simulink model "Me492CasterM2V1"  (R2026b)
settings: Solver=ode4  StopTime=4  FixedStep=solver_step_s
InitFcn:
  | addpath(fileparts(fileparts(get_param(bdroot,'FileName')))); m2_model_init(bdroot);
model workspace (MAT data in the model file):
  caster_contact_enabled = 1
  command_sample_dt_s = 0.01
  initial_state = [-0.08; 0; 0; 0; 0; 0; 0; 0; 0; 0; 0; 0; 0]
  p_vector = [16; 0.6; 0.45; 0.0015; 0.0045; 0.00045; -0.08; 0; 0.12; 0.075; 0.38; 0.04; 0.05; -0.18; 0; 9.81; 0.6; 0.6; 300; 600; 200; 250; 0.008; 0.012; 0.00025; 0.0001; 0.004; 0.006; 0.1; 0.08; 0.002; 0.12]
  solver_step_s = 0.0005
  torque_array = [0 0.01 0.02 0.03 0.04 0.05 0.06 0.07 0.08 0.09 0.1 0.11 ... (1203 elements, 401x3)]
settings Model: Creator=lelfs  LastModifiedBy=lelfs
settings DataIOCC: SaveOutput=off  SignalLogging=off

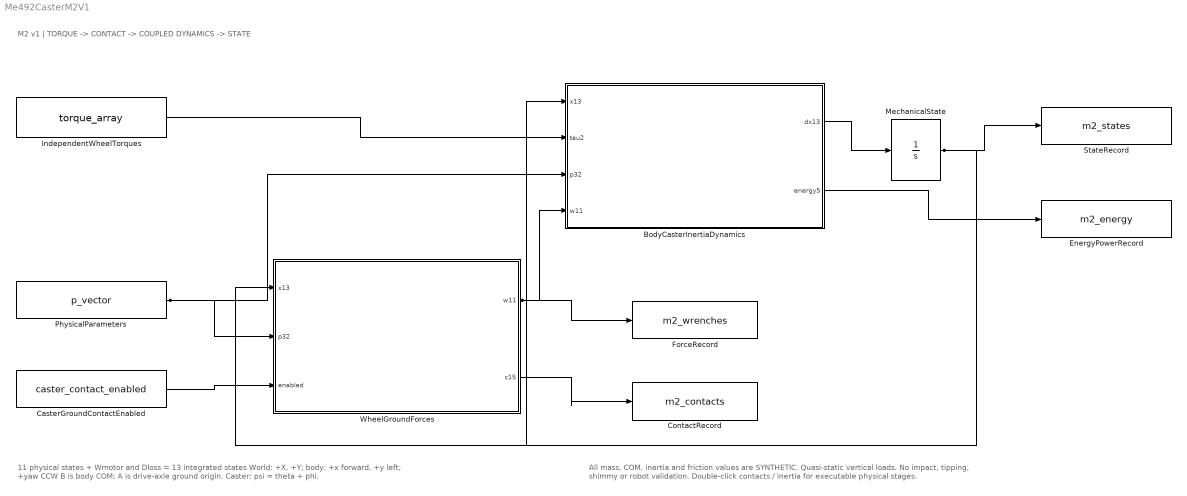
== system Me492CasterM2V1 ==
  note: M2 v1 | TORQUE -> CONTACT -> COUPLED DYNAMICS -> STATE
  note: 11 physical states + Wmotor and Dloss = 13 integrated states
      | World: +X, +Y; body: +x forward, +y left; +yaw CCW
      | B is body COM; A is drive-axle ground origin. Caster: psi = theta + phi.
  note: All mass, COM, inertia and friction values are SYNTHETIC.
      | Quasi-static vertical loads. No impact, tipping, shimmy or robot validation.
      | Double-click contacts / inertia for executable physical stages.
  BodyCasterInertiaDynamics : Subsystem
      mask Display: disp('M * nuDot + bias = Q');port_label('input',1,'x13');port_label('input',2,'tauL/R [N m]');port_label('input',3,'p32 [SI]');port_label('input',4,'F / tau');port_label('output',1,'dx13/dt');port_label('output',2,'energy / power');
  CasterGroundContactEnabled : Constant  Value=caster_contact_enabled
  ContactRecord : ToWorkspace  VariableName=m2_contacts  SaveFormat=Timeseries  SampleTime=-1
  EnergyPowerRecord : ToWorkspace  VariableName=m2_energy  SaveFormat=Timeseries  SampleTime=-1
  ForceRecord : ToWorkspace  VariableName=m2_wrenches  SaveFormat=Timeseries  SampleTime=-1
  IndependentWheelTorques : FromWorkspace  VariableName=torque_array  SampleTime=command_sample_dt_s  Interpolate=off  OutputAfterFinalValue=Holding final value
  MechanicalState : Integrator  InitialCondition=initial_state
  PhysicalParameters : Constant  Value=p_vector
  StateRecord : ToWorkspace  VariableName=m2_states  SaveFormat=Timeseries  SampleTime=-1
  WheelGroundForces : Subsystem
      mask Display: disp('Loads -> slip -> passive contact');port_label('input',1,'x13');port_label('input',2,'p32 [SI]');port_label('input',3,'enabled');port_label('output',1,'F / tau');port_label('output',2,'slip / N');
  wires:
  IndependentWheelTorques/1 -> BodyCasterInertiaDynamics/2(tau2)
  PhysicalParameters/1 -> WheelGroundForces/2(p32), BodyCasterInertiaDynamics/3(p32)
  CasterGroundContactEnabled/1 -> WheelGroundForces/3(enabled)
  WheelGroundForces/1(w11) -> BodyCasterInertiaDynamics/4(w11), ForceRecord/1
  BodyCasterInertiaDynamics/1(dx13) -> MechanicalState/1
  MechanicalState/1 -> StateRecord/1, WheelGroundForces/1(x13), BodyCasterInertiaDynamics/1(x13)
  BodyCasterInertiaDynamics/2(energy5) -> EnergyPowerRecord/1
  WheelGroundForces/2(c15) -> ContactRecord/1

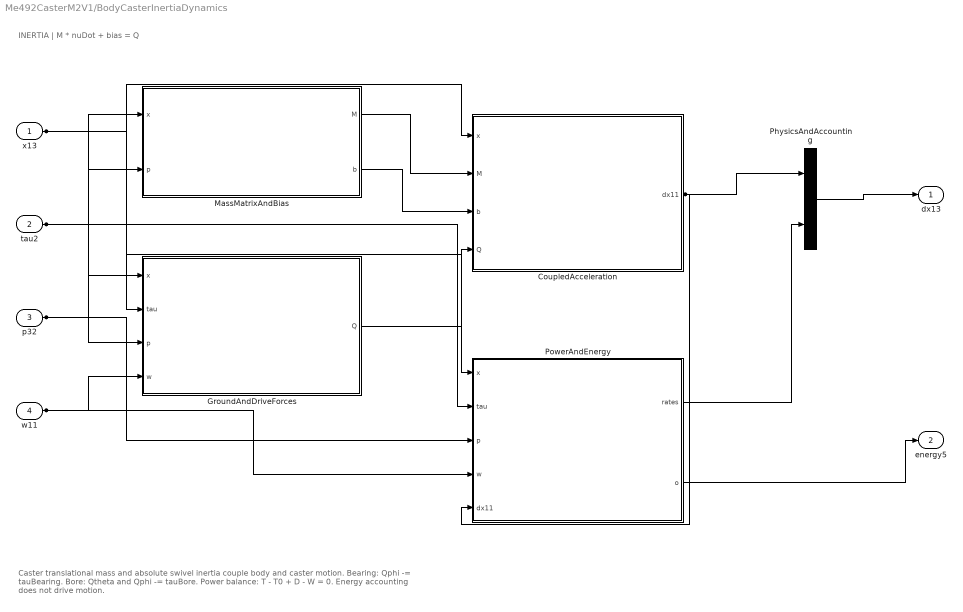
== system Me492CasterM2V1/BodyCasterInertiaDynamics ==
  note: INERTIA | M * nuDot + bias = Q
  note: Caster translational mass and absolute swivel inertia couple body and caster motion.
      | Bearing: Qphi -= tauBearing. Bore: Qtheta and Qphi -= tauBore.
      | Power balance: T - T0 + D - W = 0. Energy accounting does not drive motion.
  x13 : Inport
  tau2 : Inport  Port=2
  p32 : Inport  Port=3
  w11 : Inport  Port=4
  CoupledAcceleration : MATLAB Function  TreatAsAtomicUnit=on
  GroundAndDriveForces : MATLAB Function  TreatAsAtomicUnit=on
  MassMatrixAndBias : MATLAB Function  TreatAsAtomicUnit=on
  PhysicsAndAccounting : Mux  Inputs=2
  PowerAndEnergy : MATLAB Function  TreatAsAtomicUnit=on
  dx13 : Outport
  energy5 : Outport  Port=2
  wires:
  x13/1 -> MassMatrixAndBias/1(x), GroundAndDriveForces/1(x), PowerAndEnergy/1(x), CoupledAcceleration/1(x)
  p32/1 -> MassMatrixAndBias/2(p), GroundAndDriveForces/3(p), PowerAndEnergy/3(p)
  tau2/1 -> GroundAndDriveForces/2(tau), PowerAndEnergy/2(tau)
  w11/1 -> GroundAndDriveForces/4(w), PowerAndEnergy/4(w)
  MassMatrixAndBias/1(M) -> CoupledAcceleration/2(M)
  MassMatrixAndBias/2(b) -> CoupledAcceleration/3(b)
  GroundAndDriveForces/1(Q) -> CoupledAcceleration/4(Q)
  CoupledAcceleration/1(dx11) -> PowerAndEnergy/5(dx11), PhysicsAndAccounting/1
  PowerAndEnergy/1(rates) -> PhysicsAndAccounting/2
  PhysicsAndAccounting/1 -> dx13/1
  PowerAndEnergy/2(o) -> energy5/1

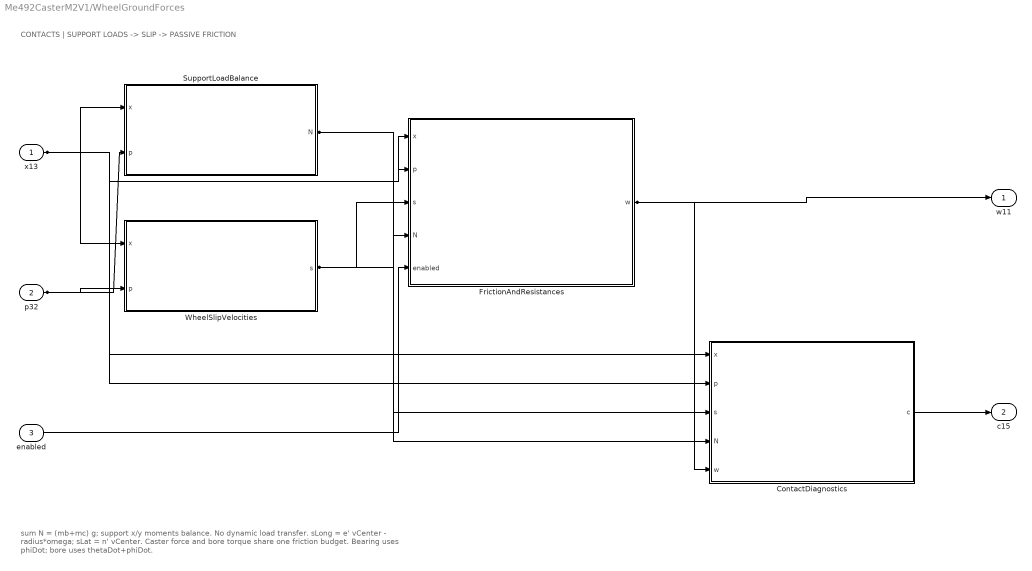
== system Me492CasterM2V1/WheelGroundForces ==
  note: CONTACTS | SUPPORT LOADS -> SLIP -> PASSIVE FRICTION
  note: sum N = (mb+mc) g; support x/y moments balance. No dynamic load transfer.
      | sLong = e' vCenter - radius*omega; sLat = n' vCenter.
      | Caster force and bore torque share one friction budget. Bearing uses phiDot; bore uses thetaDot+phiDot.
  x13 : Inport
  p32 : Inport  Port=2
  enabled : Inport  Port=3
  ContactDiagnostics : MATLAB Function  TreatAsAtomicUnit=on
  FrictionAndResistances : MATLAB Function  TreatAsAtomicUnit=on
  SupportLoadBalance : MATLAB Function  TreatAsAtomicUnit=on
  WheelSlipVelocities : MATLAB Function  TreatAsAtomicUnit=on
  w11 : Outport
  c15 : Outport  Port=2
  wires:
  x13/1 -> SupportLoadBalance/1(x), WheelSlipVelocities/1(x), FrictionAndResistances/1(x), ContactDiagnostics/1(x)
  p32/1 -> SupportLoadBalance/2(p), WheelSlipVelocities/2(p), FrictionAndResistances/2(p), ContactDiagnostics/2(p)
  WheelSlipVelocities/1(s) -> FrictionAndResistances/3(s), ContactDiagnostics/3(s)
  SupportLoadBalance/1(N) -> FrictionAndResistances/4(N), ContactDiagnostics/4(N)
  enabled/1 -> FrictionAndResistances/5(enabled)
  FrictionAndResistances/1(w) -> ContactDiagnostics/5(w), w11/1
  ContactDiagnostics/1(c) -> c15/1

== matlab function Me492CasterM2V1/WheelGroundForces/WheelSlipVelocities ==
  data: x input; s output; p input
function s=slip(x,p)
%#codegen
s=m2_slip(x,p);
end

== matlab function Me492CasterM2V1/WheelGroundForces/SupportLoadBalance ==
  data: x input; N output; p input
function N=loads(x,p)
%#codegen
N=m2_support_loads(x,p);
end

== matlab function Me492CasterM2V1/WheelGroundForces/FrictionAndResistances ==
  data: x input; w output; p input; s input; N input; enabled input
function w=forces(x,p,s,N,enabled)
%#codegen
w=m2_friction(x,p,s,N,enabled);
end

== matlab function Me492CasterM2V1/WheelGroundForces/ContactDiagnostics ==
  data: x input; c output; p input; s input; N input; w input
function c=diagnostics(x,p,s,N,w)
%#codegen
c=m2_contact_diagnostics(x,p,s,N,w);
end

== matlab function Me492CasterM2V1/BodyCasterInertiaDynamics/MassMatrixAndBias ==
  data: x input; M output; p input; b output
function [M,b]=inertia(x,p)
%#codegen
[M,b]=m2_mass_terms(x,p);
end

== matlab function Me492CasterM2V1/BodyCasterInertiaDynamics/GroundAndDriveForces ==
  data: x input; Q output; tau input; p input; w input
function Q=generalized(x,tau,p,w)
%#codegen
Q=m2_generalized_forces(x,tau(:),p,w);
end

== matlab function Me492CasterM2V1/BodyCasterInertiaDynamics/CoupledAcceleration ==
  data: x input; dx11 output; M input; b input; Q input
function dx11=motion(x,M,b,Q)
%#codegen
dx11=m2_motion_rhs(x,M,b,Q);
end

== matlab function Me492CasterM2V1/BodyCasterInertiaDynamics/PowerAndEnergy ==
  data: x input; rates output; tau input; p input; w input; dx11 input; o output
function [rates,o]=power(x,tau,p,w,dx11)
%#codegen
[rates,o]=m2_energy_power(x,tau(:),p,w,dx11);
end
